simulink model "tcp_ip"  (R2021b)
settings: Solver=ode5  StartTime=0.0  StopTime=inf  FixedStep=1/20  RelTol=1e-3
PreLoadFcn:
  | mbxruntime.callbacks.PreLoadFcn(bdroot);
PostLoadFcn:
  | mbxruntime.callbacks.PostLoadFcn(bdroot);
InitFcn:
  | mbxruntime.callbacks.InitFcn(bdroot);
StartFcn:
  | mbxruntime.callbacks.StartFcn(bdroot);
StopFcn:
  | mbxruntime.callbacks.StopFcn(bdroot);
model workspace: external: MAT-File .\kea_demo_0218_cs_hws.mat (data not in the file)
undefined symbols (not defined in the file): DiscIntNeverNeededParam, kea_demo_0218_cs_1d5c9b61e8e009e5, kea_demo_0218_cs_4669f259e7287783, kea_demo_0218_cs_87ee11d7829c0052, kea_demo_0218_cs_Audi_A3_1_Dynamics_Simple_initialPitch, kea_demo_0218_cs_Audi_A3_1_Dynamics_Simple_initialRoll, kea_demo_0218_cs_Audi_A3_1_Dynamics_Simple_initialX, kea_demo_0218_cs_Audi_A3_1_Dynamics_Simple_initialY, kea_demo_0218_cs_Audi_A3_1_Dynamics_Simple_initialYaw, kea_demo_0218_cs_Audi_A3_1_Dynamics_Simple_initialZ, kea_demo_0218_cs_Audi_A3_1_PathFollower_Preview_1_PathUniqueID, kea_demo_0218_cs_Roewe_550_S_Sedan_1_Dynamics_Simple_initialX, kea_demo_0218_cs_Roewe_550_S_Sedan_1_Dynamics_Simple_initialY, kea_demo_0218_cs_Roewe_550_S_Sedan_1_Dynamics_Simple_initialYaw, kea_demo_0218_cs_Roewe_550_S_Sedan_1_Dynamics_Simple_initialZ, mbxruntime, warningInitialVelocity, x0
libraries: simulink x56, simulink_extras x18, instrumentlib x2
(part 3 of 7)

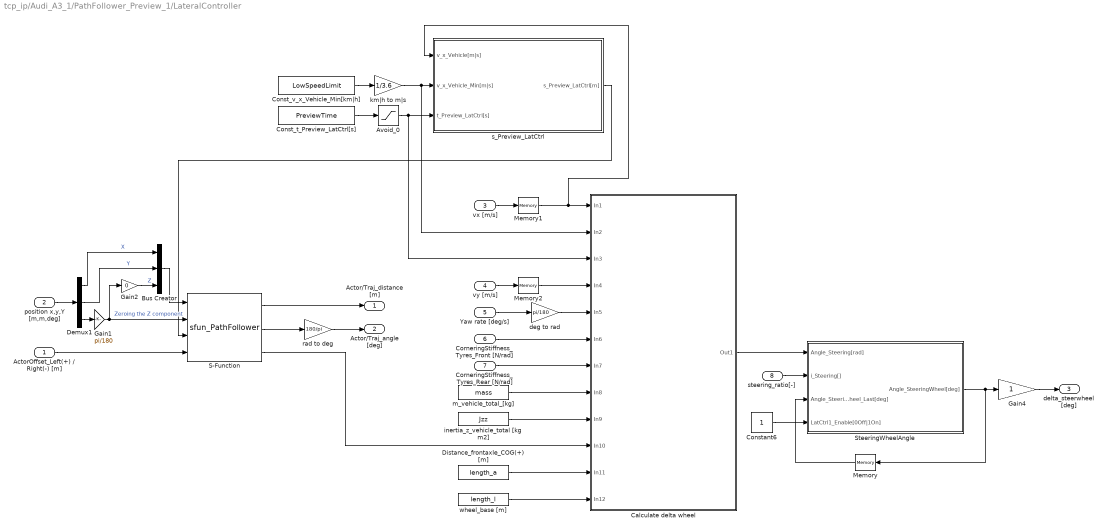
== system tcp_ip/Audi_A3_1/PathFollower_Preview_1/LateralController ==
  ActorOffset_Left(+) / Right(-) [m] : Inport
  position x,y,Y [m,m,deg] : Inport  Port=2
  vx [m/s] : Inport  Port=3
  vy [m/s] : Inport  Port=4
  Yaw rate [deg/s] : Inport  Port=5
  CorneringStiffness_Tyres_Front [N/rad] : Inport  Port=6
  CorneringStiffness_Tyres_Rear [N/rad] : Inport  Port=7
  steering_ratio[-] : Inport  Port=8
  Avoid_0 : Saturate  UpperLimit=1000  LowerLimit=0.1
  Bus Creator : BusCreator  Inputs='X','Y','Z'  OutDataTypeStr=Bus: PRESCAN_XYZ_DATA
  Calculate delta wheel : Subsystem
      mask Display:
      | port_label('input', 1, 'v_x_vehicle [m/s]')
      | port_label('input', 2, 'v_x_vehicle_Min [m/s]')
      | port_label('input', 3, 't_Preview_LatCtrl [s]')
      | port_label('input', 4, 'v_y_vehicle [m/s]')
      | port_label('input', 5, 'yawrate_vehicle [rad/sec]')
      | port_label('input', 6, 'CorneringStiffness_Tyres_Front [N/rad]')
      | port_label('input', 7, 'CorneringStiffness_Tyres_Rear [N/rad]')
      | port_label('input', 8, 'm_vehicle_total [kg]')
      | port_label('input', 9, 'inertia_z_vehicle_total [kg m2]')
      | port_label('input', 10, 'e_Lat [m]')
      | port_label('input', 11, 'Distance_frontaxle_COG(+) [m]')
      | port_label('input', 12, 'wheel_base [m]')
      | port_label('output', 1, 'delta_wheel [rad]')
  Const_t_Preview_LatCtrl[s] : Constant  Value=PreviewTime  SampleTime=CSSampleTime
  Const_v_x_Vehicle_Min[km|h] : Constant  Value=LowSpeedLimit  SampleTime=CSSampleTime
  Constant6 : Constant  SampleTime=CSSampleTime
  Demux1 : Demux  Outputs=3
  Distance_frontaxle_COG(+) [m] : Constant  Value=length_a  SampleTime=CSSampleTime
  Gain1 : Gain  Gain=pi/180
  Gain2 : Gain  Gain=0
  Gain4 : Gain
  Memory : Memory  InheritSampleTime=on
  Memory1 : Memory  InheritSampleTime=on
  Memory2 : Memory  InheritSampleTime=on
  S-Function : S-Function  FunctionName=sfun_PathFollower  Parameters=PathUniqueID,-1  SFunctionDeploymentMode=off  EnableBusSupport=off
  SteeringWheelAngle : Subsystem
  deg to rad : Gain  Gain=pi/180
  inertia_z_vehicle_total [kg m2] : Constant  Value=Jzz  SampleTime=CSSampleTime
  km|h to m|s : Gain  Gain=1/3.6
  m_vehicle_total_[kg] : Constant  Value=mass  SampleTime=CSSampleTime
  rad to deg : Gain  Gain=180/pi
  s_Preview_LatCtrl : Subsystem
  wheel_base [m] : Constant  Value=length_l  SampleTime=CSSampleTime
  Actor/Traj_distance [m] : Outport  VectorParamsAs1DForOutWhenUnconnected=off
  Actor/Traj_angle [deg] : Outport  Port=2  VectorParamsAs1DForOutWhenUnconnected=off
  delta_steerwheel [deg] : Outport  Port=3  VectorParamsAs1DForOutWhenUnconnected=off
  wires:
  Gain2/1 -> Bus Creator/3  "Z"
  Bus Creator/1 -> S-Function/1
  Demux1/2 -> Bus Creator/2  "Y"
  Demux1/1 -> Bus Creator/1  "X"
  s_Preview_LatCtrl/1(s_Preview_LatCtrl[m]) -> S-Function/3
  rad to deg/1 -> Actor/Traj_angle [deg]/1
  km|h to m|s/1 -> Calculate delta wheel/2(In2), s_Preview_LatCtrl/2(v_x_Vehicle_Min[m|s])
  ActorOffset_Left(+) / Right(-) [m]/1 -> S-Function/4
  S-Function/2 -> rad to deg/1
  S-Function/1 -> Actor/Traj_distance [m]/1
  Calculate delta wheel/1(Out1) -> SteeringWheelAngle/1(Angle_Steering[rad])
  vx [m/s]/1 -> Memory1/1
  vy [m/s]/1 -> Memory2/1
  CorneringStiffness_Tyres_Front [N/rad]/1 -> Calculate delta wheel/6(In6)
  m_vehicle_total_[kg]/1 -> Calculate delta wheel/8(In8)
  inertia_z_vehicle_total [kg m2]/1 -> Calculate delta wheel/9(In9)
  steering_ratio[-]/1 -> SteeringWheelAngle/2(i_Steering[])
  SteeringWheelAngle/1(Angle_SteeringWheel[deg]) -> Gain4/1, Memory/1
  Memory/1 -> SteeringWheelAngle/3(Angle_SteeringWheel_Last[deg])
  Constant6/1 -> SteeringWheelAngle/4(LatCtrl1_Enable[0Off|1On])
  Avoid_0/1 -> Calculate delta wheel/3(In3), s_Preview_LatCtrl/3(t_Preview_LatCtrl[s])
  Const_v_x_Vehicle_Min[km|h]/1 -> km|h to m|s/1
  Const_t_Preview_LatCtrl[s]/1 -> Avoid_0/1
  Gain4/1 -> delta_steerwheel [deg]/1
  Distance_frontaxle_COG(+) [m]/1 -> Calculate delta wheel/11(In11)
  CorneringStiffness_Tyres_Rear [N/rad]/1 -> Calculate delta wheel/7(In7)
  Yaw rate [deg/s]/1 -> deg to rad/1
  deg to rad/1 -> Calculate delta wheel/5(In5)
  Gain1/1 -> Gain2/1, S-Function/2  "Zeroing the Z component"
  Demux1/3 -> Gain1/1
  position x,y,Y [m,m,deg]/1 -> Demux1/1
  wheel_base [m]/1 -> Calculate delta wheel/12(In12)
  S-Function/3 -> Calculate delta wheel/10(In10)
  Memory1/1 -> Calculate delta wheel/1(In1), s_Preview_LatCtrl/1(v_x_Vehicle[m|s])
  Memory2/1 -> Calculate delta wheel/4(In4)

== system tcp_ip/Audi_A3_1/PathFollower_Preview_1/LongitudinalController ==
  v_actual [m/s] : Inport
  Desired Velocity [m/s] : Inport  Port=2
  Initial Velocity [m/s] : Inport  Port=3
  Check_Initial_Velocity : Subsystem
  Demux : Demux  Outputs=3
  GearNormal : Constant
  "GearNormal " : Constant
  If Desired Velocity = 0 : Subsystem  TreatAsAtomicUnit=on
  If Desired Velocity ~= 0 : Subsystem  TreatAsAtomicUnit=on
  Memory External IC : Subsystem
  Merge : Merge
  Mux : Mux  Inputs=3
  Mux2 : Mux  Inputs=3
  Sum4 : Sum  Inputs=|+-
  if : If  IfExpression=u1 == 0  SampleTime=CSSampleTime
  throttle [%] : Outport  VectorParamsAs1DForOutWhenUnconnected=off
  brake pressure [bar] : Outport  Port=2  VectorParamsAs1DForOutWhenUnconnected=off
  v0 [m/s] : Outport  Port=3  VectorParamsAs1DForOutWhenUnconnected=off
  Auto_GearShift : Outport  Port=4  VectorParamsAs1DForOutWhenUnconnected=off
  wires:
  v_actual [m/s]/1 -> Check_Initial_Velocity/1(" v_actual_[m|s]"), Memory External IC/1(u)
  Memory External IC/1(y) -> Sum4/2
  Sum4/1 -> If Desired Velocity ~= 0/2(Desired Velocity [m/s])
  Desired Velocity [m/s]/1 -> if/1, Sum4/1
  Initial Velocity [m/s]/1 -> Check_Initial_Velocity/2(Initial_Velocity_[m|s]), Memory External IC/2(IC), v0 [m/s]/1
  GearNormal/1 -> If Desired Velocity = 0/1(In1)
  Merge/1 -> Demux/1
  If Desired Velocity = 0/1(throttle [%]) -> Mux/1
  If Desired Velocity = 0/2(brake pressure [bar]) -> Mux/2
  Mux2/1 -> Merge/2
  Mux/1 -> Merge/1
  Demux/1 -> throttle [%]/1
  Demux/2 -> brake pressure [bar]/1
  Demux/3 -> Auto_GearShift/1
  "GearNormal "/1 -> If Desired Velocity ~= 0/1(In1)
  If Desired Velocity = 0/3(Auto_GearShift) -> Mux/3
  if/2 -> If Desired Velocity ~= 0/Action
  if/1 -> If Desired Velocity = 0/Action
  If Desired Velocity ~= 0/1(throttle [%]) -> Mux2/1
  If Desired Velocity ~= 0/2(brake pressure [bar]) -> Mux2/2
  If Desired Velocity ~= 0/3(Auto_GearShift) -> Mux2/3

== system tcp_ip/Audi_A3_1/SELF_Demux/compas converter ==
  rotz [rad] : Inport
  cart2compas : Subsystem
  rad2deg : Gain  Gain=180/pi
  heading [deg] : Outport  VectorParamsAs1DForOutWhenUnconnected=off
  wires:
  rad2deg/1 -> cart2compas/1(Angle [deg])
  rotz [rad]/1 -> rad2deg/1
  cart2compas/1(heading [deg]) -> heading [deg]/1

== system tcp_ip/Roewe_550_S_Sedan_1/AIR_2_Demux/Activate_Switch ==
  BeamID : Inport
  Heading : Inport  Port=2
  Constant : Constant  Value=0
  Product1 : Product  RndMeth=Zero
  Relational Operator : RelationalOperator  Operator=~=  OutDataTypeStr=boolean  RndMeth=Nearest
  On/Off : Outport  VectorParamsAs1DForOutWhenUnconnected=off
  wires:
  Heading/1 -> Product1/2
  Product1/1 -> On/Off/1
  BeamID/1 -> Relational Operator/2
  Relational Operator/1 -> Product1/1
  Constant/1 -> Relational Operator/1

== system tcp_ip/Roewe_550_S_Sedan_1/AIR_2_Demux/Signal2ArrayOfSignals1 ==
  note: Initial state of Previous vector block
      | set to zeros(VECTORLENGTH,1)
  note: Set mask parameter VECTORLENGTH
      |  to MAXMESSAGES
  LoopIndex : Inport
  Element : Inport  Port=2
  Assignment : Assignment  IndexOptions=Index vector (port)  Indices=1  OutputSizes=1
  Previous vector : Memory  InitialCondition=zeros(VECTORLENGTH,1)  InheritSampleTime=on
  ArrayofElements : Outport  VectorParamsAs1DForOutWhenUnconnected=off
  wires:
  Assignment/1 -> Previous vector/1, ArrayofElements/1
  Previous vector/1 -> Assignment/1
  LoopIndex/1 -> Assignment/3
  Element/1 -> Assignment/2

== system tcp_ip/Roewe_550_S_Sedan_1/AIR_2_Demux/Signal2ArrayOfSignals2 ==
  note: Initial state of Previous vector block
      | set to zeros(VECTORLENGTH,1)
  note: Set mask parameter VECTORLENGTH
      |  to MAXMESSAGES
  LoopIndex : Inport
  Element : Inport  Port=2
  Assignment : Assignment  IndexOptions=Index vector (port)  Indices=1  OutputSizes=1
  Previous vector : Memory  InitialCondition=zeros(VECTORLENGTH,1)  InheritSampleTime=on
  ArrayofElements : Outport  VectorParamsAs1DForOutWhenUnconnected=off
  wires:
  Assignment/1 -> Previous vector/1, ArrayofElements/1
  Previous vector/1 -> Assignment/1
  LoopIndex/1 -> Assignment/3
  Element/1 -> Assignment/2

== system tcp_ip/Roewe_550_S_Sedan_1/AIR_2_Demux/Signal2ArrayOfSignals3 ==
  note: Initial state of Previous vector block
      | set to zeros(VECTORLENGTH,1)
  note: Set mask parameter VECTORLENGTH
      |  to MAXMESSAGES
  LoopIndex : Inport
  Element : Inport  Port=2
  Assignment : Assignment  IndexOptions=Index vector (port)  Indices=1  OutputSizes=1
  Previous vector : Memory  InitialCondition=zeros(VECTORLENGTH,1)  InheritSampleTime=on
  ArrayofElements : Outport  VectorParamsAs1DForOutWhenUnconnected=off
  wires:
  Assignment/1 -> Previous vector/1, ArrayofElements/1
  Previous vector/1 -> Assignment/1
  LoopIndex/1 -> Assignment/3
  Element/1 -> Assignment/2

== system tcp_ip/Roewe_550_S_Sedan_1/AIR_2_Demux/Signal2ArrayOfSignals4 ==
  note: Initial state of Previous vector block
      | set to zeros(VECTORLENGTH,1)
  note: Set mask parameter VECTORLENGTH
      |  to MAXMESSAGES
  LoopIndex : Inport
  Element : Inport  Port=2
  Assignment : Assignment  IndexOptions=Index vector (port)  Indices=1  OutputSizes=1
  Previous vector : Memory  InitialCondition=zeros(VECTORLENGTH,1)  InheritSampleTime=on
  ArrayofElements : Outport  VectorParamsAs1DForOutWhenUnconnected=off
  wires:
  Assignment/1 -> Previous vector/1, ArrayofElements/1
  Previous vector/1 -> Assignment/1
  LoopIndex/1 -> Assignment/3
  Element/1 -> Assignment/2

== system tcp_ip/Roewe_550_S_Sedan_1/AIR_2_Demux/Signal2ArrayOfSignals5 ==
  note: Initial state of Previous vector block
      | set to zeros(VECTORLENGTH,1)
  note: Set mask parameter VECTORLENGTH
      |  to MAXMESSAGES
  LoopIndex : Inport
  Element : Inport  Port=2
  Assignment : Assignment  IndexOptions=Index vector (port)  Indices=1  OutputSizes=1
  Previous vector : Memory  InitialCondition=zeros(VECTORLENGTH,1)  InheritSampleTime=on
  ArrayofElements : Outport  VectorParamsAs1DForOutWhenUnconnected=off
  wires:
  Assignment/1 -> Previous vector/1, ArrayofElements/1
  Previous vector/1 -> Assignment/1
  LoopIndex/1 -> Assignment/3
  Element/1 -> Assignment/2

== system tcp_ip/Roewe_550_S_Sedan_1/AIR_2_Demux/Signal2ArrayOfSignals6 ==
  note: Initial state of Previous vector block
      | set to zeros(VECTORLENGTH,1)
  note: Set mask parameter VECTORLENGTH
      |  to MAXMESSAGES
  LoopIndex : Inport
  Element : Inport  Port=2
  Assignment : Assignment  IndexOptions=Index vector (port)  Indices=1  OutputSizes=1
  Previous vector : Memory  InitialCondition=zeros(VECTORLENGTH,1)  InheritSampleTime=on
  ArrayofElements : Outport  VectorParamsAs1DForOutWhenUnconnected=off
  wires:
  Assignment/1 -> Previous vector/1, ArrayofElements/1
  Previous vector/1 -> Assignment/1
  LoopIndex/1 -> Assignment/3
  Element/1 -> Assignment/2

== system tcp_ip/Roewe_550_S_Sedan_1/AIR_2_Demux/Signal2ArrayOfSignals7 ==
  note: Initial state of Previous vector block
      | set to zeros(VECTORLENGTH,1)
  note: Set mask parameter VECTORLENGTH
      |  to MAXMESSAGES
  LoopIndex : Inport
  Element : Inport  Port=2
  Assignment : Assignment  IndexOptions=Index vector (port)  Indices=1  OutputSizes=1
  Previous vector : Memory  InitialCondition=zeros(VECTORLENGTH,1)  InheritSampleTime=on
  ArrayofElements : Outport  VectorParamsAs1DForOutWhenUnconnected=off
  wires:
  Assignment/1 -> Previous vector/1, ArrayofElements/1
  Previous vector/1 -> Assignment/1
  LoopIndex/1 -> Assignment/3
  Element/1 -> Assignment/2

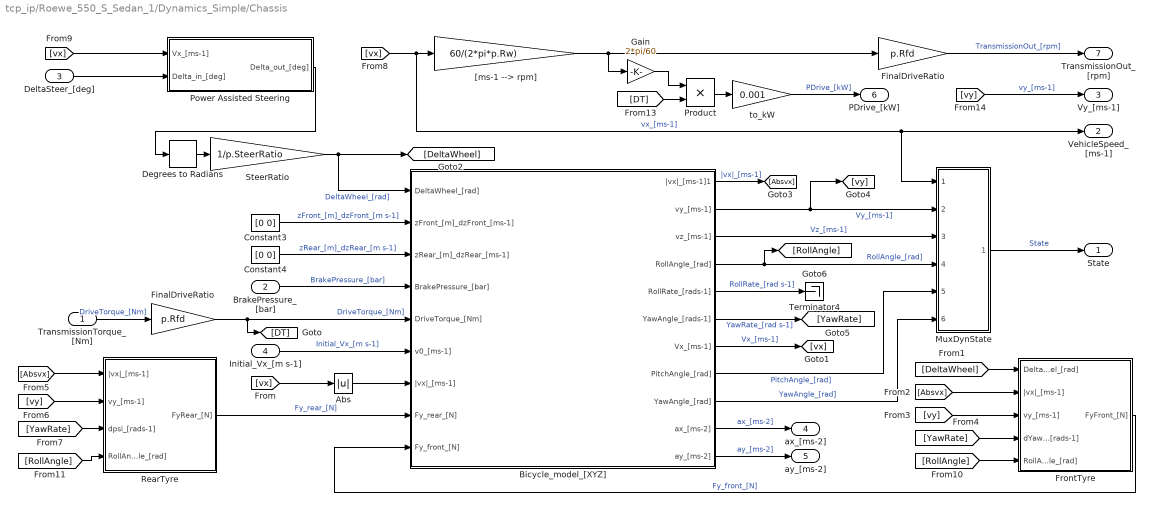
== system tcp_ip/Roewe_550_S_Sedan_1/Dynamics_Simple/Chassis ==
  TransmissionTorque_[Nm] : Inport
  BrakePressure_[bar] : Inport  Port=2
  DeltaSteer_[deg] : Inport  Port=3
  Initial_Vx_[m s-1] : Inport  Port=4
  Abs : Abs
  Bicycle_model_[XYZ] : Subsystem
      mask Display: image(imread('Bicycle_model.png'));
  Constant3 : Constant  Value=[0 0]
  Constant4 : Constant  Value=[0 0]
  Degrees to Radians : simulink_extras/Transformations/Degrees to Radians
  FinalDriveRatio : Gain  Gain=p.Rfd  SaturateOnIntegerOverflow=on  OutDataTypeStr=Inherit: Same as input  ParamDataTypeStr=Inherit: Same as input
  "FinalDriveRatio " : Gain  Gain=p.Rfd  SaturateOnIntegerOverflow=on  OutDataTypeStr=Inherit: Same as input  ParamDataTypeStr=Inherit: Same as input
  FrontTyre : Subsystem
      mask Display: image(imread('Tyre.png'));
  Gain : Gain  Gain=2*pi/60
  MuxDynState : Subsystem
  Power Assisted Steering : Subsystem
  Product : Product  RndMeth=Zero
  RearTyre : Subsystem
      mask Display: image(imread('Tyre.png'));
  SteerRatio : Gain  Gain=1/p.SteerRatio
  Terminator4 : Terminator
  "[ms-1 --> rpm]" : Gain  Gain=60/(2*pi*p.Rw)  SaturateOnIntegerOverflow=on  OutDataTypeStr=Inherit: Same as input  ParamDataTypeStr=Inherit: Same as input
  to_kW : Gain  Gain=0.001
  State : Outport  VectorParamsAs1DForOutWhenUnconnected=off
  VehicleSpeed_[ms-1] : Outport  Port=2  VectorParamsAs1DForOutWhenUnconnected=off
  Vy_[ms-1] : Outport  Port=3  VectorParamsAs1DForOutWhenUnconnected=off
  ax_[ms-2] : Outport  Port=4  VectorParamsAs1DForOutWhenUnconnected=off
  ay_[ms-2] : Outport  Port=5  VectorParamsAs1DForOutWhenUnconnected=off
  PDrive_[kW] : Outport  Port=6  VectorParamsAs1DForOutWhenUnconnected=off
  TransmissionOut_[rpm] : Outport  Port=7  VectorParamsAs1DForOutWhenUnconnected=off
  wires:
  [vy] -> Vy_[ms-1]/1  "vy_[ms-1]"
  to_kW/1 -> PDrive_[kW]/1  "PDrive_[kW]"
  Gain/1 -> Product/1
  Bicycle_model_[XYZ]/10(ax_[ms-2]) -> ax_[ms-2]/1  "ax_[ms-2]"
  Product/1 -> to_kW/1
  [DT] -> Product/2
  Bicycle_model_[XYZ]/11(ay_[ms-2]) -> ay_[ms-2]/1  "ay_[ms-2]"
  Abs/1 -> Bicycle_model_[XYZ]/7(|vx|_[ms-1])
  Degrees to Radians/1 -> SteerRatio/1
  [vx] -> Abs/1
  SteerRatio/1 -> [DeltaWheel], Bicycle_model_[XYZ]/1(DeltaWheel_[rad])  "DeltaWheel_[rad]"
  TransmissionTorque_[Nm]/1 -> "FinalDriveRatio "/1  "DriveTorque_[Nm]"
  RearTyre/1(FyRear_[N]) -> Bicycle_model_[XYZ]/8(Fy_rear_[N])  "Fy_rear_[N]"
  FrontTyre/1(FyFront_[N]) -> Bicycle_model_[XYZ]/9(Fy_front_[N])  "Fy_front_[N]"
  Bicycle_model_[XYZ]/1(|vx|_[ms-1]1) -> [Absvx]  "|vx|_[ms-1]"
  Bicycle_model_[XYZ]/2(vy_[ms-1]) -> [vy], MuxDynState/2(vy [ms-1])  "Vy_[ms-1]"
  Bicycle_model_[XYZ]/4(RollAngle_[rad]) -> MuxDynState/4(R [rad]), [RollAngle]  "RollAngle_[rad]"
  Bicycle_model_[XYZ]/6(YawAngle_[rads-1]) -> [YawRate]  "YawRate_[rad s-1]"
  Bicycle_model_[XYZ]/7(Vx_[ms-1]) -> [vx]  "Vx_[ms-1]"
  [DeltaWheel] -> FrontTyre/1(DeltaWheel_[rad])
  [Absvx] -> FrontTyre/2(|vx|_[ms-1])
  [vy] -> FrontTyre/3(vy_[ms-1])
  [YawRate] -> FrontTyre/4(dYawAngle_[rads-1])
  [Absvx] -> RearTyre/1(|vx|_[ms-1])
  [vy] -> RearTyre/2(vy_[ms-1])
  [YawRate] -> RearTyre/3(dpsi_[rads-1])
  Bicycle_model_[XYZ]/3(vz_[ms-1]) -> MuxDynState/3(vz [ms-1])  "Vz_[ms-1]"
  Bicycle_model_[XYZ]/8(PitchAngle_[rad]) -> MuxDynState/5(P [rad])  "PitchAngle_[rad]"
  Bicycle_model_[XYZ]/9(YawAngle_[rad]) -> MuxDynState/6(Y [rad])  "YawAngle_[rad]"
  "[ms-1 --> rpm]"/1 -> Gain/1, FinalDriveRatio/1
  FinalDriveRatio/1 -> TransmissionOut_[rpm]/1  "TransmissionOut_[rpm]"
  [vx] -> "[ms-1 --> rpm]"/1, VehicleSpeed_[ms-1]/1, MuxDynState/1(vx [ms-1])  "vx_[ms-1]"
  [vx] -> Power Assisted Steering/1(Vx_[ms-1])
  DeltaSteer_[deg]/1 -> Power Assisted Steering/2(Delta_in_[deg])
  Power Assisted Steering/1(Delta_out_[deg]) -> Degrees to Radians/1
  [RollAngle] -> FrontTyre/5(RollAngle_[rad])
  [RollAngle] -> RearTyre/4(RollAngle_[rad])
  Constant3/1 -> Bicycle_model_[XYZ]/2(zFront_[m]_dzFront_[ms-1])  "zFront_[m]_dzFront_[m s-1]"
  Constant4/1 -> Bicycle_model_[XYZ]/3(zRear_[m]_dzRear_[ms-1])  "zRear_[m]_dzRear_[m s-1]"
  BrakePressure_[bar]/1 -> Bicycle_model_[XYZ]/4(BrakePressure_[bar])  "BrakePressure_[bar]"
  "FinalDriveRatio "/1 -> Bicycle_model_[XYZ]/5(DriveTorque_[Nm]), [DT]  "DriveTorque_[Nm]"
  Initial_Vx_[m s-1]/1 -> Bicycle_model_[XYZ]/6(v0_[ms-1])  "Initial_Vx_[m s-1]"
  Bicycle_model_[XYZ]/5(RollRate_[rads-1]) -> Terminator4/1  "RollRate_[rad s-1]"
  MuxDynState/1(State) -> State/1  "State"

== system tcp_ip/Roewe_550_S_Sedan_1/Dynamics_Simple/Engine ==
  ImpellerTorque_[Nm] : Inport
  Throttle_[%] : Inport  Port=2
  Configurable Subsystem : Subsystem  Variant=on  VariantControlMode=label  LabelModeActiveChoice=Continuous
      settings: AttributesFormatString=%<BlockChoice>  OpenFcn=BringToFront(gcb);
  Configurable Subsystem1 : Subsystem  Variant=on  VariantControlMode=label  LabelModeActiveChoice=Continuous
      settings: AttributesFormatString=%<BlockChoice>  OpenFcn=BringToFront(gcb);
  EngineTorque : Lookup2D  RowIndex=p.thvec  ColumnIndex=p.nevec  Table=p.emap  InputSameDT=on
  Gain : Gain  Gain=2*pi/60
  Product : Product  RndMeth=Zero
  Sum : Sum  Inputs=-+  InputSameDT=on  SaturateOnIntegerOverflow=on  OutDataTypeStr=Inherit: Same as first input
  engine + impeller inertia : Gain  Gain=1/p.Iei  SaturateOnIntegerOverflow=on  OutDataTypeStr=Inherit: Same as input  ParamDataTypeStr=Inherit: Same as input
  rad|sec2rpm : Gain  Gain=60/2/pi  SaturateOnIntegerOverflow=on  OutDataTypeStr=Inherit: Same as input  ParamDataTypeStr=Inherit: Same as input
  to_kW : Gain  Gain=0.001
  nEngine_[rpm] : Outport  InitialOutput=0  VectorParamsAs1DForOutWhenUnconnected=off
  PEngine_[kW] : Outport  Port=2  InitialOutput=0  VectorParamsAs1DForOutWhenUnconnected=off
  wires:
  rad|sec2rpm/1 -> nEngine_[rpm]/1, EngineTorque/2, Gain/1  "rpm"
  engine + impeller inertia/1 -> Configurable Subsystem1/1(In1)  "rads-2"
  EngineTorque/1 -> Sum/2, Product/2
  Sum/1 -> engine + impeller inertia/1
  Configurable Subsystem1/1(Out1) -> rad|sec2rpm/1  "rads-1"
  Throttle_[%]/1 -> Configurable Subsystem/1(In1)
  ImpellerTorque_[Nm]/1 -> Sum/1
  Configurable Subsystem/1(Out1) -> EngineTorque/1
  Product/1 -> to_kW/1
  Gain/1 -> Product/1
  to_kW/1 -> PEngine_[kW]/1

== system tcp_ip/Roewe_550_S_Sedan_1/Dynamics_Simple/Gear: Auto Manual ==
  note: 0; Auto = on // Manual =off
      | 1; Auto = off // Manual =on
  Auto_Manual : Inport
  Manual_Gear : Inport  Port=2
  Auto_Gear : Inport  Port=3
  If : If  IfExpression=u1 == 0
  If Action Subsystem : Subsystem  TreatAsAtomicUnit=on
  If Action Subsystem1 : Subsystem  TreatAsAtomicUnit=on
  Merge : Merge
  Gear : Outport  VectorParamsAs1DForOutWhenUnconnected=off
  wires:
  If Action Subsystem/1(Out1) -> Merge/1
  Auto_Gear/1 -> If Action Subsystem/1(In1)
  If/1 -> If Action Subsystem/Action
  Merge/1 -> Gear/1
  If Action Subsystem1/1(Out1) -> Merge/2
  Manual_Gear/1 -> If Action Subsystem1/1(In1)
  If/2 -> If Action Subsystem1/Action
  Auto_Manual/1 -> If/1

== system tcp_ip/Roewe_550_S_Sedan_1/Dynamics_Simple/ShiftLogic ==
  Throttle_[%] : Inport
  GearNr_[-] : Inport  Port=2
  Auto_GearShift : Inport  Port=3
  VehSpeed_[ms-1] : Inport  Port=4
  Add2 : Sum
  Data Type Conversion1 : DataTypeConversion  OutDataTypeStr=double
  Detect Increase1 : simulink/Logic and Bit Operations/Detect Increase  vinit=0.0  OutDataTypeStr=uint8
  Detect Increase : Subsystem
  Gear limitation : Saturate  UpperLimit=p.maxGear  LowerLimit=1
  Gear limitation while shifting : Saturate  UpperLimit=p.maxGear  LowerLimit=1
  GearNeutral : Constant  Value=0
  GearReverse : Constant  Value=-1
  "IC, gear = 1" : Memory  InitialCondition=1  InheritSampleTime=on
  If Action Neutral : Subsystem  TreatAsAtomicUnit=on
  If Action Normal : Subsystem  TreatAsAtomicUnit=on
  If Action Reverse : Subsystem  TreatAsAtomicUnit=on
  Memory : Memory  InheritSampleTime=on
  Merge : Merge  Inputs=3
  Relational Operator : RelationalOperator  OutDataTypeStr=boolean  RndMeth=Nearest
  Relational Operator1 : RelationalOperator  Operator=<=  OutDataTypeStr=boolean  RndMeth=Nearest
  Shift_Down time : Delay  DelayLength=p.ShiftDown_fac
  Shift_Up time : Delay  DelayLength=p.ShiftUp_fac
  Sum : Sum  Inputs=+-
  interp_down : Lookup2D  RowIndex=p.downth  ColumnIndex=[1:p.maxGear]  Table=p.downtab  LookUpMeth=Interpolation-Use End Values  InputSameDT=on
  interp_up : Lookup2D  RowIndex=p.upth  ColumnIndex=[1:p.maxGear]  Table=p.uptab  LookUpMeth=Interpolation-Use End Values  InputSameDT=on
  reverse/neutral/normal gear : If  IfExpression=u1 == 0  ElseIfExpressions=u1 < 0
  to_ms-1 : Gain  Gain=1/3.6
  "to_ms-1 " : Gain  Gain=1/3.6
  GearNr : Outport  VectorParamsAs1DForOutWhenUnconnected=off
  wires:
  Auto_GearShift/1 -> reverse/neutral/normal gear/1
  "IC, gear = 1"/1 -> If Action Normal/1(In1)
  Merge/1 -> GearNr/1
  If Action Reverse/1(Out1) -> Merge/2
  If Action Neutral/1(Out1) -> Merge/1
  If Action Normal/1(Out1) -> Merge/3
  reverse/neutral/normal gear/3 -> If Action Normal/Action
  reverse/neutral/normal gear/1 -> If Action Neutral/Action
  reverse/neutral/normal gear/2 -> If Action Reverse/Action
  GearReverse/1 -> If Action Reverse/1(In1)
  GearNeutral/1 -> If Action Neutral/1(In1)
  Shift_Down time/1 -> Sum/2
  Shift_Up time/1 -> Sum/1
  Detect Increase/1(Out1) -> Shift_Up time/1
  Data Type Conversion1/1 -> Shift_Down time/1
  Detect Increase1/1 -> Data Type Conversion1/1
  Sum/1 -> Add2/1
  Memory/1 -> Add2/2  "GearNr_[-]"
  Add2/1 -> Gear limitation while shifting/1
  Gear limitation while shifting/1 -> "IC, gear = 1"/1, Memory/1  "GearNr_[-]"
  Throttle_[%]/1 -> interp_down/1, interp_up/1
  Relational Operator/1 -> Detect Increase/2(In2)
  Relational Operator1/1 -> Detect Increase1/1
  interp_down/1 -> "to_ms-1 "/1
  VehSpeed_[ms-1]/1 -> Relational Operator/1, Relational Operator1/1
  interp_up/1 -> to_ms-1/1
  Gear limitation/1 -> interp_down/2, interp_up/2, Detect Increase/1(GearNr_[-])
  GearNr_[-]/1 -> Gear limitation/1
  to_ms-1/1 -> Relational Operator/2
  "to_ms-1 "/1 -> Relational Operator1/2

== system tcp_ip/Roewe_550_S_Sedan_1/Dynamics_Simple/State2Bus1 ==
  State : Inport  SampleTime=TimeStep
  Bus Creator : BusCreator  Inputs=15  OutDataTypeStr=Bus: PRESCAN_STATEACTUATORDATA  NonVirtualBus=on
  Constant : Constant  Value=0
  Demux : Demux  Outputs=15
  Mux : Mux  Inputs=3
  Mux1 : Mux  Inputs=3
  Mux2 : Mux  Inputs=3
  iniBODYAngles wrtVEH [rad] : Constant  Value=Roll0  SampleTime=TimeStep
  iniBODYAngles wrtVEH [rad]1 : Constant  Value=Pitch0  SampleTime=TimeStep
  iniVEHAngles wrtGLOB [rad] : Constant  Value=Yaw0  SampleTime=TimeStep
  iniVEHposition wrtGLOB [m] : Constant  Value=x0  SampleTime=TimeStep
  iniVEHposition wrtGLOB [m]1 : Constant  Value=y0  SampleTime=TimeStep
  iniVEHposition wrtGLOB [m]2 : Constant  Value=z0  SampleTime=TimeStep
  state2FullState : Subsystem  mask(PreScan Demux Block:){}
  StateBus : Outport  OutDataTypeStr=Bus: PRESCAN_STATEACTUATORDATA  VectorParamsAs1DForOutWhenUnconnected=off
  wires:
  Mux2/1 -> state2FullState/4(iniVEH Angles wrt GLOB axis system [deg])
  iniVEHAngles wrtGLOB [rad]/1 -> Mux2/3
  Mux1/1 -> state2FullState/3(iniBODY Angles wrt VEH axis system [deg])
  Constant/1 -> Mux2/1, Mux2/2, Mux1/3
  iniBODYAngles wrtVEH [rad]1/1 -> Mux1/2
  iniBODYAngles wrtVEH [rad]/1 -> Mux1/1
  Mux/1 -> state2FullState/2(ini VEHpos wrt GLOB axis system [m])
  iniVEHposition wrtGLOB [m]2/1 -> Mux/3
  iniVEHposition wrtGLOB [m]/1 -> Mux/1
  iniVEHposition wrtGLOB [m]1/1 -> Mux/2
  Demux/15 -> Bus Creator/15  "AngularVelocityYaw"
  Demux/14 -> Bus Creator/14  "AngularVelocityPitch"
  Demux/13 -> Bus Creator/13  "AngularVelocityRoll"
  Demux/12 -> Bus Creator/12  "OrientationYaw"
  Demux/11 -> Bus Creator/11  "OrientationPitch"
  Demux/10 -> Bus Creator/10  "OrientationRoll"
  Demux/9 -> Bus Creator/9  "AccelerationZ"
  Demux/8 -> Bus Creator/8  "AccelerationY"
  Demux/7 -> Bus Creator/7  "AccelerationX"
  Demux/6 -> Bus Creator/6  "VelocityZ"
  Demux/5 -> Bus Creator/5  "VelocityY"
  Demux/4 -> Bus Creator/4  "VelocityX"
  Demux/3 -> Bus Creator/3  "PositionZ"
  Demux/2 -> Bus Creator/2  "PositionY"
  Demux/1 -> Bus Creator/1  "PositionX"
  state2FullState/1(State) -> Demux/1
  State/1 -> state2FullState/1(dx,dy,dz [m/s] R,P,Y [rad])
  Bus Creator/1 -> StateBus/1

== system tcp_ip/Roewe_550_S_Sedan_1/Dynamics_Simple/Transmission ==
  nEngine_[rpm] : Inport
  GearNr_[-] : Inport  Port=2
  n_TransmissionOut_[rpm] : Inport  Port=3
  Torque_Converter : Subsystem
      mask Display: image(imread('TorqueConverter.png'));
  Transmission_Ratio : Subsystem
  Viscous coupling : Lookup  InputValues=[-5:0.1:5]*p.m/4  Table=p.m/4*tanh([-5:0.1:5])
  ImpellerTorque_[Nm] : Outport  InitialOutput=0  VectorParamsAs1DForOutWhenUnconnected=off
  TransmissionTorque_[Nm] : Outport  Port=2  InitialOutput=0  VectorParamsAs1DForOutWhenUnconnected=off
  wires:
  Torque_Converter/2(TurbineTorque_[Nm]) -> Viscous coupling/1  "Converter_Torque_[Nm]"
  Transmission_Ratio/2(nTransmissionIn_[rpm]) -> Torque_Converter/2(nTransmission_[rpm])
  nEngine_[rpm]/1 -> Torque_Converter/1(nEngine_[rpm])
  GearNr_[-]/1 -> Transmission_Ratio/2(GearNr_[-]), Torque_Converter/3(Gear nr)
  n_TransmissionOut_[rpm]/1 -> Transmission_Ratio/3(nTransmissionOut_[rpm])
  Torque_Converter/1(ImpellerTorque_[Nm]) -> ImpellerTorque_[Nm]/1
  Transmission_Ratio/1(tTransmissionOut_[Nm]) -> TransmissionTorque_[Nm]/1
  Viscous coupling/1 -> Transmission_Ratio/1(tTransmissionIn_[Nm])

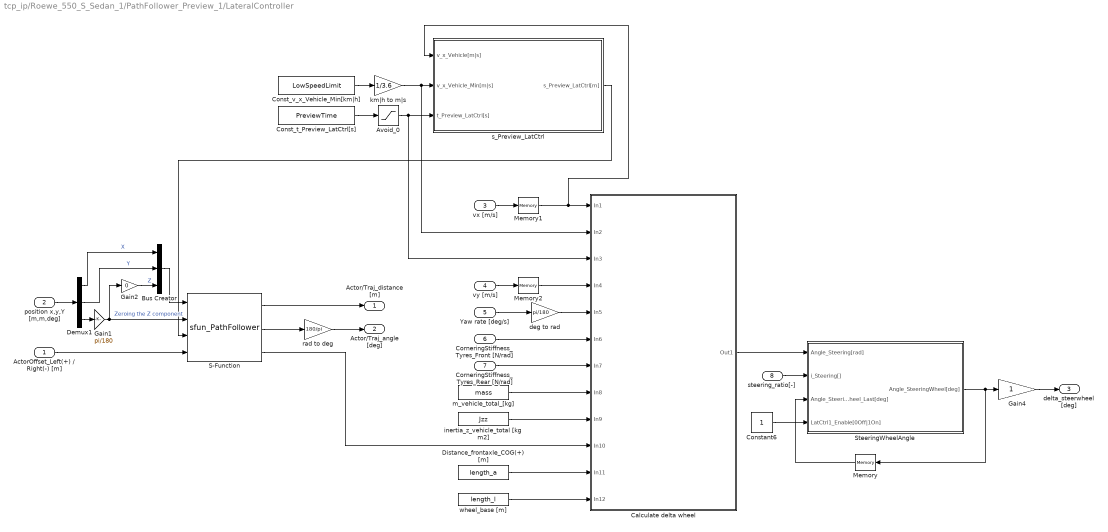
== system tcp_ip/Roewe_550_S_Sedan_1/PathFollower_Preview_1/LateralController ==
  ActorOffset_Left(+) / Right(-) [m] : Inport
  position x,y,Y [m,m,deg] : Inport  Port=2
  vx [m/s] : Inport  Port=3
  vy [m/s] : Inport  Port=4
  Yaw rate [deg/s] : Inport  Port=5
  CorneringStiffness_Tyres_Front [N/rad] : Inport  Port=6
  CorneringStiffness_Tyres_Rear [N/rad] : Inport  Port=7
  steering_ratio[-] : Inport  Port=8
  Avoid_0 : Saturate  UpperLimit=1000  LowerLimit=0.1
  Bus Creator : BusCreator  Inputs='X','Y','Z'  OutDataTypeStr=Bus: PRESCAN_XYZ_DATA
  Calculate delta wheel : Subsystem
      mask Display:
      | port_label('input', 1, 'v_x_vehicle [m/s]')
      | port_label('input', 2, 'v_x_vehicle_Min [m/s]')
      | port_label('input', 3, 't_Preview_LatCtrl [s]')
      | port_label('input', 4, 'v_y_vehicle [m/s]')
      | port_label('input', 5, 'yawrate_vehicle [rad/sec]')
      | port_label('input', 6, 'CorneringStiffness_Tyres_Front [N/rad]')
      | port_label('input', 7, 'CorneringStiffness_Tyres_Rear [N/rad]')
      | port_label('input', 8, 'm_vehicle_total [kg]')
      | port_label('input', 9, 'inertia_z_vehicle_total [kg m2]')
      | port_label('input', 10, 'e_Lat [m]')
      | port_label('input', 11, 'Distance_frontaxle_COG(+) [m]')
      | port_label('input', 12, 'wheel_base [m]')
      | port_label('output', 1, 'delta_wheel [rad]')
  Const_t_Preview_LatCtrl[s] : Constant  Value=PreviewTime  SampleTime=CSSampleTime
  Const_v_x_Vehicle_Min[km|h] : Constant  Value=LowSpeedLimit  SampleTime=CSSampleTime
  Constant6 : Constant  SampleTime=CSSampleTime
  Demux1 : Demux  Outputs=3
  Distance_frontaxle_COG(+) [m] : Constant  Value=length_a  SampleTime=CSSampleTime
  Gain1 : Gain  Gain=pi/180
  Gain2 : Gain  Gain=0
  Gain4 : Gain
  Memory : Memory  InheritSampleTime=on
  Memory1 : Memory  InheritSampleTime=on
  Memory2 : Memory  InheritSampleTime=on
  S-Function : S-Function  FunctionName=sfun_PathFollower  Parameters=PathUniqueID,-1  SFunctionDeploymentMode=off  EnableBusSupport=off
  SteeringWheelAngle : Subsystem
  deg to rad : Gain  Gain=pi/180
  inertia_z_vehicle_total [kg m2] : Constant  Value=Jzz  SampleTime=CSSampleTime
  km|h to m|s : Gain  Gain=1/3.6
  m_vehicle_total_[kg] : Constant  Value=mass  SampleTime=CSSampleTime
  rad to deg : Gain  Gain=180/pi
  s_Preview_LatCtrl : Subsystem
  wheel_base [m] : Constant  Value=length_l  SampleTime=CSSampleTime
  Actor/Traj_distance [m] : Outport  VectorParamsAs1DForOutWhenUnconnected=off
  Actor/Traj_angle [deg] : Outport  Port=2  VectorParamsAs1DForOutWhenUnconnected=off
  delta_steerwheel [deg] : Outport  Port=3  VectorParamsAs1DForOutWhenUnconnected=off
  wires:
  Gain2/1 -> Bus Creator/3  "Z"
  Bus Creator/1 -> S-Function/1
  Demux1/2 -> Bus Creator/2  "Y"
  Demux1/1 -> Bus Creator/1  "X"
  s_Preview_LatCtrl/1(s_Preview_LatCtrl[m]) -> S-Function/3
  rad to deg/1 -> Actor/Traj_angle [deg]/1
  km|h to m|s/1 -> Calculate delta wheel/2(In2), s_Preview_LatCtrl/2(v_x_Vehicle_Min[m|s])
  ActorOffset_Left(+) / Right(-) [m]/1 -> S-Function/4
  S-Function/2 -> rad to deg/1
  S-Function/1 -> Actor/Traj_distance [m]/1
  Calculate delta wheel/1(Out1) -> SteeringWheelAngle/1(Angle_Steering[rad])
  vx [m/s]/1 -> Memory1/1
  vy [m/s]/1 -> Memory2/1
  CorneringStiffness_Tyres_Front [N/rad]/1 -> Calculate delta wheel/6(In6)
  m_vehicle_total_[kg]/1 -> Calculate delta wheel/8(In8)
  inertia_z_vehicle_total [kg m2]/1 -> Calculate delta wheel/9(In9)
  steering_ratio[-]/1 -> SteeringWheelAngle/2(i_Steering[])
  SteeringWheelAngle/1(Angle_SteeringWheel[deg]) -> Gain4/1, Memory/1
  Memory/1 -> SteeringWheelAngle/3(Angle_SteeringWheel_Last[deg])
  Constant6/1 -> SteeringWheelAngle/4(LatCtrl1_Enable[0Off|1On])
  Avoid_0/1 -> Calculate delta wheel/3(In3), s_Preview_LatCtrl/3(t_Preview_LatCtrl[s])
  Const_v_x_Vehicle_Min[km|h]/1 -> km|h to m|s/1
  Const_t_Preview_LatCtrl[s]/1 -> Avoid_0/1
  Gain4/1 -> delta_steerwheel [deg]/1
  Distance_frontaxle_COG(+) [m]/1 -> Calculate delta wheel/11(In11)
  CorneringStiffness_Tyres_Rear [N/rad]/1 -> Calculate delta wheel/7(In7)
  Yaw rate [deg/s]/1 -> deg to rad/1
  deg to rad/1 -> Calculate delta wheel/5(In5)
  Gain1/1 -> Gain2/1, S-Function/2  "Zeroing the Z component"
  Demux1/3 -> Gain1/1
  position x,y,Y [m,m,deg]/1 -> Demux1/1
  wheel_base [m]/1 -> Calculate delta wheel/12(In12)
  S-Function/3 -> Calculate delta wheel/10(In10)
  Memory1/1 -> Calculate delta wheel/1(In1), s_Preview_LatCtrl/1(v_x_Vehicle[m|s])
  Memory2/1 -> Calculate delta wheel/4(In4)

== system tcp_ip/Roewe_550_S_Sedan_1/PathFollower_Preview_1/LongitudinalController ==
  v_actual [m/s] : Inport
  Desired Velocity [m/s] : Inport  Port=2
  Initial Velocity [m/s] : Inport  Port=3
  Check_Initial_Velocity : Subsystem
  Demux : Demux  Outputs=3
  GearNormal : Constant
  "GearNormal " : Constant
  If Desired Velocity = 0 : Subsystem  TreatAsAtomicUnit=on
  If Desired Velocity ~= 0 : Subsystem  TreatAsAtomicUnit=on
  Memory External IC : Subsystem
  Merge : Merge
  Mux : Mux  Inputs=3
  Mux2 : Mux  Inputs=3
  Sum4 : Sum  Inputs=|+-
  if : If  IfExpression=u1 == 0  SampleTime=CSSampleTime
  throttle [%] : Outport  VectorParamsAs1DForOutWhenUnconnected=off
  brake pressure [bar] : Outport  Port=2  VectorParamsAs1DForOutWhenUnconnected=off
  v0 [m/s] : Outport  Port=3  VectorParamsAs1DForOutWhenUnconnected=off
  Auto_GearShift : Outport  Port=4  VectorParamsAs1DForOutWhenUnconnected=off
  wires:
  v_actual [m/s]/1 -> Check_Initial_Velocity/1(" v_actual_[m|s]"), Memory External IC/1(u)
  Memory External IC/1(y) -> Sum4/2
  Sum4/1 -> If Desired Velocity ~= 0/2(Desired Velocity [m/s])
  Desired Velocity [m/s]/1 -> if/1, Sum4/1
  Initial Velocity [m/s]/1 -> Check_Initial_Velocity/2(Initial_Velocity_[m|s]), Memory External IC/2(IC), v0 [m/s]/1
  GearNormal/1 -> If Desired Velocity = 0/1(In1)
  Merge/1 -> Demux/1
  If Desired Velocity = 0/1(throttle [%]) -> Mux/1
  If Desired Velocity = 0/2(brake pressure [bar]) -> Mux/2
  Mux2/1 -> Merge/2
  Mux/1 -> Merge/1
  Demux/1 -> throttle [%]/1
  Demux/2 -> brake pressure [bar]/1
  Demux/3 -> Auto_GearShift/1
  "GearNormal "/1 -> If Desired Velocity ~= 0/1(In1)
  If Desired Velocity = 0/3(Auto_GearShift) -> Mux/3
  if/2 -> If Desired Velocity ~= 0/Action
  if/1 -> If Desired Velocity = 0/Action
  If Desired Velocity ~= 0/1(throttle [%]) -> Mux2/1
  If Desired Velocity ~= 0/2(brake pressure [bar]) -> Mux2/2
  If Desired Velocity ~= 0/3(Auto_GearShift) -> Mux2/3

== system tcp_ip/Roewe_550_S_Sedan_1/SELF_Demux/compas converter ==
  rotz [rad] : Inport
  cart2compas : Subsystem
  rad2deg : Gain  Gain=180/pi
  heading [deg] : Outport  VectorParamsAs1DForOutWhenUnconnected=off
  wires:
  rad2deg/1 -> cart2compas/1(Angle [deg])
  rotz [rad]/1 -> rad2deg/1
  cart2compas/1(heading [deg]) -> heading [deg]/1

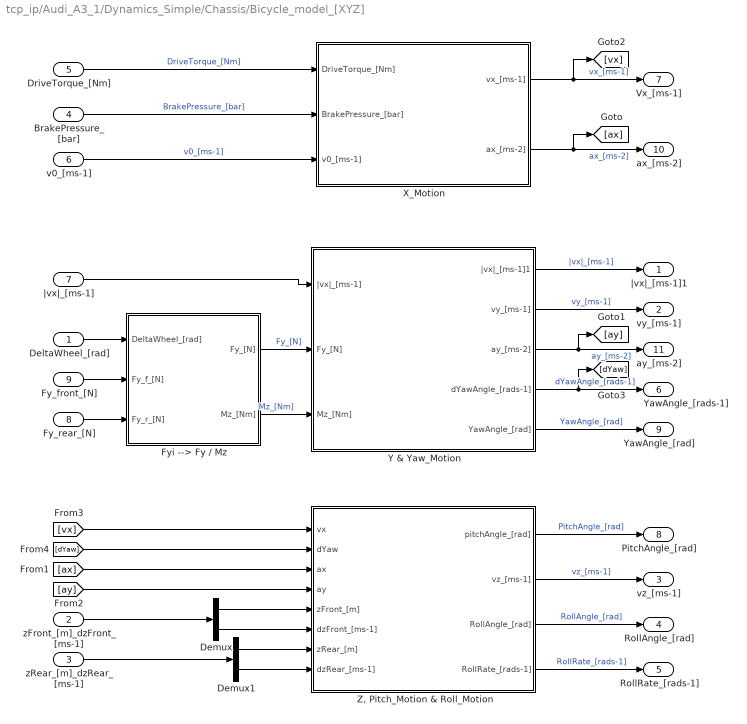
== system tcp_ip/Audi_A3_1/Dynamics_Simple/Chassis/Bicycle_model_[XYZ] ==
  DeltaWheel_[rad] : Inport
  zFront_[m]_dzFront_[ms-1] : Inport  Port=2  PortDimensions=2
  zRear_[m]_dzRear_[ms-1] : Inport  Port=3  PortDimensions=2
  BrakePressure_[bar] : Inport  Port=4
  DriveTorque_[Nm] : Inport  Port=5
  v0_[ms-1] : Inport  Port=6
  |vx|_[ms-1] : Inport  Port=7
  Fy_rear_[N] : Inport  Port=8
  Fy_front_[N] : Inport  Port=9
  Demux : Demux  Outputs=2
  Demux1 : Demux  Outputs=2
  Fyi --> Fy / Mz : Subsystem
  X_Motion : Subsystem
  Y & Yaw_Motion : Subsystem
  "Z, Pitch_Motion & Roll_Motion" : Subsystem
  |vx|_[ms-1]1 : Outport  VectorParamsAs1DForOutWhenUnconnected=off
  vy_[ms-1] : Outport  Port=2  VectorParamsAs1DForOutWhenUnconnected=off
  vz_[ms-1] : Outport  Port=3  VectorParamsAs1DForOutWhenUnconnected=off
  RollAngle_[rad] : Outport  Port=4  VectorParamsAs1DForOutWhenUnconnected=off
  RollRate_[rads-1] : Outport  Port=5  VectorParamsAs1DForOutWhenUnconnected=off
  YawAngle_[rads-1] : Outport  Port=6  VectorParamsAs1DForOutWhenUnconnected=off
  Vx_[ms-1] : Outport  Port=7  VectorParamsAs1DForOutWhenUnconnected=off
  PitchAngle_[rad] : Outport  Port=8  VectorParamsAs1DForOutWhenUnconnected=off
  YawAngle_[rad] : Outport  Port=9  VectorParamsAs1DForOutWhenUnconnected=off
  ax_[ms-2] : Outport  Port=10  VectorParamsAs1DForOutWhenUnconnected=off
  ay_[ms-2] : Outport  Port=11  VectorParamsAs1DForOutWhenUnconnected=off
  wires:
  Fyi --> Fy / Mz/1(Fy_[N]) -> Y & Yaw_Motion/2(Fy_[N])  "Fy_[N]"
  Fyi --> Fy / Mz/2(Mz_[Nm]) -> Y & Yaw_Motion/3(Mz_[Nm])  "Mz_[Nm]"
  Y & Yaw_Motion/1(|vx|_[ms-1]1) -> |vx|_[ms-1]1/1  "|vx|_[ms-1]"
  Y & Yaw_Motion/2(vy_[ms-1]) -> vy_[ms-1]/1  "vy_[ms-1]"
  Y & Yaw_Motion/5(YawAngle_[rad]) -> YawAngle_[rad]/1  "YawAngle_[rad]"
  v0_[ms-1]/1 -> X_Motion/3(v0_[ms-1])  "v0_[ms-1]"
  BrakePressure_[bar]/1 -> X_Motion/2(BrakePressure_[bar])  "BrakePressure_[bar]"
  DriveTorque_[Nm]/1 -> X_Motion/1(DriveTorque_[Nm])  "DriveTorque_[Nm]"
  X_Motion/2(ax_[ms-2]) -> ax_[ms-2]/1, [ax]  "ax_[ms-2]"
  X_Motion/1(vx_[ms-1]) -> Vx_[ms-1]/1, [vx]  "vx_[ms-1]"
  [ax] -> "Z, Pitch_Motion & Roll_Motion"/3(ax)
  Demux/1 -> "Z, Pitch_Motion & Roll_Motion"/5(zFront_[m])
  Demux/2 -> "Z, Pitch_Motion & Roll_Motion"/6(dzFront_[ms-1])
  Demux1/1 -> "Z, Pitch_Motion & Roll_Motion"/7(zRear_[m])
  Demux1/2 -> "Z, Pitch_Motion & Roll_Motion"/8(dzRear_[ms-1])
  zRear_[m]_dzRear_[ms-1]/1 -> Demux1/1
  zFront_[m]_dzFront_[ms-1]/1 -> Demux/1
  "Z, Pitch_Motion & Roll_Motion"/2(vz_[ms-1]) -> vz_[ms-1]/1  "vz_[ms-1]"
  DeltaWheel_[rad]/1 -> Fyi --> Fy / Mz/1(DeltaWheel_[rad])
  Fy_front_[N]/1 -> Fyi --> Fy / Mz/2(Fy_f_[N])
  Fy_rear_[N]/1 -> Fyi --> Fy / Mz/3(Fy_r_[N])
  |vx|_[ms-1]/1 -> Y & Yaw_Motion/1(|vx|_[ms-1])
  Y & Yaw_Motion/3(ay_[ms-2]) -> [ay], ay_[ms-2]/1  "ay_[ms-2]"
  [ay] -> "Z, Pitch_Motion & Roll_Motion"/4(ay)
  "Z, Pitch_Motion & Roll_Motion"/3(RollAngle_[rad]) -> RollAngle_[rad]/1  "RollAngle_[rad]"
  "Z, Pitch_Motion & Roll_Motion"/4(RollRate_[rads-1]) -> RollRate_[rads-1]/1  "RollRate_[rads-1]"
  [dYaw] -> "Z, Pitch_Motion & Roll_Motion"/2(dYaw)
  [vx] -> "Z, Pitch_Motion & Roll_Motion"/1(vx)
  Y & Yaw_Motion/4(dYawAngle_[rads-1]) -> YawAngle_[rads-1]/1, [dYaw]  "dYawAngle_[rads-1]"
  "Z, Pitch_Motion & Roll_Motion"/1(pitchAngle_[rad]) -> PitchAngle_[rad]/1  "PitchAngle_[rad]"

== system tcp_ip/Audi_A3_1/Dynamics_Simple/Chassis/FrontTyre ==
  note: alpha limiter
      | [-1 ... 1]
  note: relax_on
      | ON: 1
      | OFF: 0
  note: MOTORCYCLE ONLY
  note: VEHICLE + MOTORCYCLE
  DeltaWheel_[rad] : Inport
  |vx|_[ms-1] : Inport  Port=2
  vy_[ms-1] : Inport  Port=3
  dYawAngle_[rads-1] : Inport  Port=4
  RollAngle_[rad] : Inport  Port=5
  AlphaFront : Subsystem
  Compare To Zero : simulink/Logic and Bit Operations/Compare To Zero  relop===  OutDataTypeStr=boolean  ZeroCross=off
  Configurable Subsystem : Subsystem  Variant=on  VariantControlMode=label  LabelModeActiveChoice=Continuous
      settings: AttributesFormatString=%<BlockChoice>  OpenFcn=BringToFront(gcb);
  Configurable Subsystem1 : Subsystem  Variant=on  VariantControlMode=label  LabelModeActiveChoice=Continuous
      settings: AttributesFormatString=%<BlockChoice>  OpenFcn=BringToFront(gcb);
  Constant : Constant  Value=p.relax_on
  Constant1 : Constant  Value=p.relax_on
  Constant2 : Constant  Value=p.VehMCSwitch
  Data Type Conversion : DataTypeConversion  OutDataTypeStr=double
  If MC : simulink/Logic and Bit Operations/Compare To Constant  relop===  const=2  OutDataTypeStr=uint8  ZeroCross=off
  K_gamma_front : Gain  Gain=p.Kgfront
  Linl : Fcn  Expr=(u(4) - u(5))/p.sigma_front*u(1)
  Linl1 : Fcn  Expr=(u(4) - u(5))/p.sigma_front*u(1)
  Mux1 : Mux  Inputs=3
  Mux2 : Mux  Inputs={3,1,1}
  Mux3 : Mux  Inputs={3,1,1}
  Prevent_instability_at_low_Vx : Subsystem
  Product : Product  RndMeth=Zero
  Sum : Sum  Inputs=|++  InputSameDT=on  SaturateOnIntegerOverflow=on  OutDataTypeStr=Inherit: Same as first input
  Sum1 : Sum  Inputs=|++
  Switch : Switch  Threshold=0.5  SaturateOnIntegerOverflow=on  InputSameDT=on
  Switch1 : Switch  Threshold=0.5  SaturateOnIntegerOverflow=on  InputSameDT=on
  alg.loop : Memory
  due to sign convention : Gain  Gain=-1  SaturateOnIntegerOverflow=on  OutDataTypeStr=Inherit: Same as input  ParamDataTypeStr=Inherit: Same as input
  front_tyre : Gain  Gain=p.Kfront
  FyFront_[N] : Outport  VectorParamsAs1DForOutWhenUnconnected=off
  wires:
  Prevent_instability_at_low_Vx/1(alpha [rad]) -> Mux2/2, Switch/3
  Sum/1 -> Prevent_instability_at_low_Vx/1(alpha[rad])  "AlphaStatFront_[rad]"
  Switch/1 -> front_tyre/1  "AlphaFront_[rad]"
  Constant/1 -> Switch/2
  Sum1/1 -> FyFront_[N]/1  "FyFront_[N]"
  Mux2/1 -> Linl/1
  Linl/1 -> Configurable Subsystem/1(In1)
  Configurable Subsystem/1(Out1) -> Mux2/3, Switch/1  "AlphaRelaxFront_[rad]"
  AlphaFront/1(Alpha) -> Sum/1
  Mux1/1 -> Prevent_instability_at_low_Vx/2(In), AlphaFront/1(In), Mux2/1, Mux3/1
  |vx|_[ms-1]/1 -> Mux1/1, Compare To Zero/1
  vy_[ms-1]/1 -> Mux1/2
  dYawAngle_[rads-1]/1 -> Mux1/3
  alg.loop/1 -> Switch1/3
  Configurable Subsystem1/1(Out1) -> Mux3/3, Switch1/1  "GammaRelaxFront_[rad]"
  Linl1/1 -> Configurable Subsystem1/1(In1)
  Mux3/1 -> Linl1/1
  Constant1/1 -> Switch1/2
  due to sign convention/1 -> alg.loop/1, Mux3/2  "GammaStatFront_[rad]"
  RollAngle_[rad]/1 -> due to sign convention/1
  front_tyre/1 -> Sum1/1
  Constant2/1 -> If MC/1
  If MC/1 -> Data Type Conversion/1
  K_gamma_front/1 -> Product/1
  Product/1 -> Sum1/2
  Data Type Conversion/1 -> Product/2
  Compare To Zero/1 -> [reset]
  [reset] -> Configurable Subsystem/2(In2)
  [reset] -> Configurable Subsystem1/2(In2)
  DeltaWheel_[rad]/1 -> Sum/2  "DeltaWheel_[rad]"
  Switch1/1 -> K_gamma_front/1  "GammaFront_[rad]"

== system tcp_ip/Audi_A3_1/Dynamics_Simple/Chassis/MuxDynState ==
  note: The position inputs are computed by the
      | integrated velocity.
  note: mode: Dynamics
      | VelVEHICLE
      | wrt VEH
  note: AnglesVEHICLE
      | wrtGLOB
  vx [ms-1] : Inport
  vy [ms-1] : Inport  Port=2
  vz [ms-1] : Inport  Port=3
  R [rad] : Inport  Port=4
  P [rad] : Inport  Port=5
  Y [rad] : Inport  Port=6
  Configurable Subsystem1 : Subsystem  Variant=on  VariantControlMode=label  LabelModeActiveChoice=Continuous  mask{IntegrationMethod=Integrator: Forward Euler}
      mask prompts: IntegrationMethod "Integration method"
      mask init:
      | discreteIntegrator = strcat(gcb,'/Discrete-Time Integrator/Discrete-Time Integrator');
      | 
      | switch IntegrationMethod
      |     case 1
      |         method = 'Integration: Forward Euler';
      |     case 2
      |         method = 'Integration: Backward Euler';
      | end
      | 
      | set_param(discreteIntegrator, 'IntegratorMethod',method);
      settings: AttributesFormatString=%<BlockChoice>  OpenFcn=BringToFront(gcb);
      mask TypeOptions IntegrationMethod: Integrator: Forward Euler | Integrator: Backward Euler
  Ground : Ground
  Ground1 : Ground
  Mux : Mux  Inputs=[3 3 3]
  Mux1 : Mux  Inputs=3
  Mux2 : Mux  Inputs=3
  Transformation_BODY2GLOBAL : Subsystem
  mux3 : Mux  Inputs=3
  State : Outport  VectorParamsAs1DForOutWhenUnconnected=off
  wires:
  Ground1/1 -> mux3/2  "pitch"
  Y [rad]/1 -> Mux2/3, mux3/3  "yaw"
  P [rad]/1 -> Mux2/2
  R [rad]/1 -> Mux2/1
  vz [ms-1]/1 -> Mux1/3
  vy [ms-1]/1 -> Mux1/2
  vx [ms-1]/1 -> Mux1/1
  Mux2/1 -> Mux/3
  Transformation_BODY2GLOBAL/1(Vvector_GLOBAL_[m/s]) -> Configurable Subsystem1/1(In1), Mux/2  "VelVEH wrt  GLOB"
  mux3/1 -> Transformation_BODY2GLOBAL/2(angles_BODYwrtGLOB_[rad])
  Ground/1 -> mux3/1  "roll"
  Mux/1 -> State/1
  Mux1/1 -> Transformation_BODY2GLOBAL/1(Vvector_BODY_[m/s])
  Configurable Subsystem1/1(Out1) -> Mux/1  "PosVEH wrt  GLOB"

== system tcp_ip/Audi_A3_1/Dynamics_Simple/Chassis/Power Assisted Steering ==
  note: MOTORCYCLE
  note: VEHICLE
  note: Reverse steering direction for negative velocities
  Vx_[ms-1] : Inport
  Delta_in_[deg] : Inport  Port=2
  Constant : Constant
  Constant1 : Constant  Value=p.VehMCSwitch
  Lookup Table : Lookup  InputValues=[0 35 45 100]  Table=[1 1 0.2 0.2]
  Multiport Switch : MultiPortSwitch  Inputs=2
  Product : Product  Inputs=3  RndMeth=Zero
  Sign : Signum
  Delta_out_[deg] : Outport  VectorParamsAs1DForOutWhenUnconnected=off
  wires:
  Vx_[ms-1]/1 -> Lookup Table/1, Sign/1
  Delta_in_[deg]/1 -> Product/3
  Constant1/1 -> Multiport Switch/1
  Constant/1 -> Multiport Switch/3
  Lookup Table/1 -> Multiport Switch/2
  Multiport Switch/1 -> Product/2
  Product/1 -> Delta_out_[deg]/1
  Sign/1 -> Product/1

== system tcp_ip/Audi_A3_1/Dynamics_Simple/Chassis/RearTyre ==
  note: alpha limiter
      | [-1 ... 1]
  note: relax_on
      | ON: 1
      | OFF: 0
  note: MOTORCYCLE ONLY
  note: VEHICLE + MOTORCYCLE
  |vx|_[ms-1] : Inport
  vy_[ms-1] : Inport  Port=2
  dpsi_[rads-1] : Inport  Port=3
  RollAngle_[rad] : Inport  Port=4
  AlphaRear : Subsystem
  Compare To Zero : simulink/Logic and Bit Operations/Compare To Zero  relop===  OutDataTypeStr=boolean  ZeroCross=off
  Configurable Subsystem : Subsystem  Variant=on  VariantControlMode=label  LabelModeActiveChoice=Continuous
      settings: AttributesFormatString=%<BlockChoice>  OpenFcn=BringToFront(gcb);
  Configurable Subsystem1 : Subsystem  Variant=on  VariantControlMode=label  LabelModeActiveChoice=Continuous
      settings: AttributesFormatString=%<BlockChoice>  OpenFcn=BringToFront(gcb);
  Constant1 : Constant  Value=p.relax_on
  Constant2 : Constant  Value=p.relax_on
  Constant3 : Constant  Value=p.VehMCSwitch
  Data Type Conversion : DataTypeConversion  OutDataTypeStr=double
  If MC : simulink/Logic and Bit Operations/Compare To Constant  relop===  const=2  OutDataTypeStr=uint8  ZeroCross=off
  K_gamma_rear : Gain  Gain=p.Kgrear
  Linl : Fcn  Expr=(u(4) - u(5))/p.sigma_rear*u(1)
  Linl1 : Fcn  Expr=(u(4) - u(5))/p.sigma_rear*u(1)
  Mux1 : Mux  Inputs=3
  Mux2 : Mux  Inputs={3,1,1}
  Mux3 : Mux  Inputs={3,1,1}
  Prevent_instability_at_low_Vx : Subsystem
  Product : Product  RndMeth=Zero
  Sum1 : Sum  Inputs=|++
  Switch1 : Switch  Threshold=0.5  SaturateOnIntegerOverflow=on  InputSameDT=on
  Switch2 : Switch  Threshold=0.5  SaturateOnIntegerOverflow=on  InputSameDT=on
  alg.loop : Memory
  due to sign convention : Gain  Gain=-1  SaturateOnIntegerOverflow=on  OutDataTypeStr=Inherit: Same as input  ParamDataTypeStr=Inherit: Same as input
  rear_tyre : Gain  Gain=p.Krear
  FyRear_[N] : Outport  VectorParamsAs1DForOutWhenUnconnected=off
  wires:
  Prevent_instability_at_low_Vx/1(alpha [rad]) -> Switch1/3, Mux2/2
  AlphaRear/1(Alpha) -> Prevent_instability_at_low_Vx/1(alpha[rad])  "AlphaStatRear_[rad]"
  Switch1/1 -> rear_tyre/1  "AlphaRear_[rad]"
  Constant1/1 -> Switch1/2
  Sum1/1 -> FyRear_[N]/1  "FyRear_[N]"
  Mux2/1 -> Linl/1
  Linl/1 -> Configurable Subsystem1/1(In1)
  Configurable Subsystem1/1(Out1) -> Mux2/3, Switch1/1  "AlphaRelaxRear_[rad]"
  Mux1/1 -> Prevent_instability_at_low_Vx/2(In), AlphaRear/1(In), Mux2/1, Mux3/1
  |vx|_[ms-1]/1 -> Mux1/1, Compare To Zero/1
  vy_[ms-1]/1 -> Mux1/2
  dpsi_[rads-1]/1 -> Mux1/3
  alg.loop/1 -> Switch2/3
  Configurable Subsystem/1(Out1) -> Mux3/3, Switch2/1  "GammaRelaxRear_[rad]"
  Linl1/1 -> Configurable Subsystem/1(In1)
  Mux3/1 -> Linl1/1
  Constant2/1 -> Switch2/2
  due to sign convention/1 -> alg.loop/1, Mux3/2  "GammaStatRear_[rad]"
  RollAngle_[rad]/1 -> due to sign convention/1
  Constant3/1 -> If MC/1
  If MC/1 -> Data Type Conversion/1
  Product/1 -> Sum1/2
  Data Type Conversion/1 -> Product/2
  K_gamma_rear/1 -> Product/1
  rear_tyre/1 -> Sum1/1
  Compare To Zero/1 -> [reset]
  [reset] -> Configurable Subsystem1/2(In2)
  [reset] -> Configurable Subsystem/2(In2)
  Switch2/1 -> K_gamma_rear/1  "GammaFront_[rad]"

== system tcp_ip/Audi_A3_1/Dynamics_Simple/Engine/Configurable Subsystem ==
  In1 : Inport
  Discrete Rate Limiter : Subsystem  VariantControl=Discrete
  Rate Limiter : Subsystem  VariantControl=Continuous
  Out1 : Outport  VectorParamsAs1DForOutWhenUnconnected=off

== system tcp_ip/Audi_A3_1/Dynamics_Simple/Engine/Configurable Subsystem1 ==
  In1 : Inport
  Discrete-Time Integrator : Subsystem  VariantControl=Discrete
  Integrator : Subsystem  VariantControl=Continuous
  Out1 : Outport  VectorParamsAs1DForOutWhenUnconnected=off

== system tcp_ip/Audi_A3_1/Dynamics_Simple/Gear: Auto Manual/If Action Subsystem ==
  In1 : Inport
  Action Port : ActionPort  PropagateVarSize=During execution  ActionPortLabel=if(u1 == 0)
  Out1 : Outport  VectorParamsAs1DForOutWhenUnconnected=off
  wires:
  In1/1 -> Out1/1

== system tcp_ip/Audi_A3_1/Dynamics_Simple/Gear: Auto Manual/If Action Subsystem1 ==
  In1 : Inport
  Action Port : ActionPort  PropagateVarSize=During execution  ActionPortLabel=else
  Out1 : Outport  VectorParamsAs1DForOutWhenUnconnected=off
  wires:
  In1/1 -> Out1/1

== system tcp_ip/Audi_A3_1/Dynamics_Simple/ShiftLogic/Detect Increase ==
  GearNr_[-] : Inport
  In2 : Inport  Port=2
  Constant : Constant
  Data Type Conversion : DataTypeConversion  OutDataTypeStr=double
  Data Type Conversion1 : DataTypeConversion  OutDataTypeStr=double
  Detect Increase : simulink/Logic and Bit Operations/Detect Increase  vinit=1  OutDataTypeStr=uint8
  If : If  NumInputs=2  IfExpression="u1==1 &  u2==1"
  If V0 higher of the from 2->3 shifting velocity : Subsystem  TreatAsAtomicUnit=on
  Merge : Merge
  Other : Subsystem  TreatAsAtomicUnit=on
  Out1 : Outport  VectorParamsAs1DForOutWhenUnconnected=off
  wires:
  If/2 -> Other/Action
  If V0 higher of the from 2->3 shifting velocity/1(Out1) -> Merge/1
  Other/1(Out1) -> Merge/2
  Detect Increase/1 -> Data Type Conversion/1
  Merge/1 -> Out1/1
  If/1 -> If V0 higher of the from 2->3 shifting velocity/Action
  Data Type Conversion1/1 -> If/2
  Data Type Conversion/1 -> If/1
  Constant/1 -> If V0 higher of the from 2->3 shifting velocity/1(In1)
  GearNr_[-]/1 -> Detect Increase/1
  In2/1 -> Data Type Conversion1/1, Other/1(In1)

== system tcp_ip/Audi_A3_1/Dynamics_Simple/ShiftLogic/If Action Neutral ==
  In1 : Inport
  Action Port : ActionPort  InitializeStates=reset  PropagateVarSize=During execution  ActionPortLabel=if(u1 == 0)
  Out1 : Outport  VectorParamsAs1DForOutWhenUnconnected=off
  wires:
  In1/1 -> Out1/1

== system tcp_ip/Audi_A3_1/Dynamics_Simple/ShiftLogic/If Action Normal ==
  In1 : Inport
  Action Port : ActionPort  InitializeStates=reset  PropagateVarSize=During execution  ActionPortLabel=else
  Out1 : Outport  VectorParamsAs1DForOutWhenUnconnected=off
  wires:
  In1/1 -> Out1/1

== system tcp_ip/Audi_A3_1/Dynamics_Simple/ShiftLogic/If Action Reverse ==
  In1 : Inport
  Action Port : ActionPort  InitializeStates=reset  PropagateVarSize=During execution  ActionPortLabel=elseif(u1 < 0)
  Out1 : Outport  VectorParamsAs1DForOutWhenUnconnected=off
  wires:
  In1/1 -> Out1/1
